simulink model "Visualization_MVP_AI"  (R2026b)
settings: Solver=ode4  StopTime=90  FixedStep=0.005
libraries: uavutilslib x1
settings Model: DataDictionary=QuadInterfaces_AI.sldd  Creator=JonathanTee  LastModifiedBy=JonathanTee

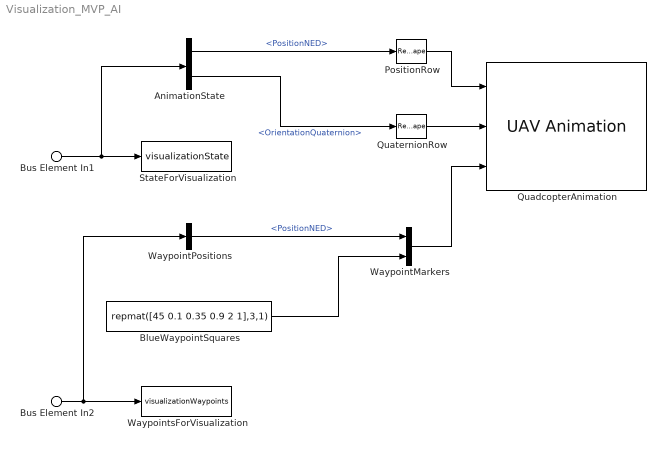
== system Visualization_MVP_AI ==
  Bus Element In1 : Inport  PortName=VehicleState
  Bus Element In2 : Inport  Port=2  PortName=WaypointTargets
  AnimationState : BusSelector  OutputSignals=PositionNED,OrientationQuaternion
  BlueWaypointSquares : Constant  Value=repmat([45 0.1 0.35 0.9 2 1],3,1)
  PositionRow : Reshape  OutputDimensionality=Row vector (2-D)
  QuadcopterAnimation : uavutilslib/UAV Animation  NumUAV=1  DynamicUAVConfig=off  UAVType=Multirotor  UAVSize=0.8  UAVColor=[0.9 0.05 0.04]  UAVTrajectoryAlpha=1  AlwaysShowAnimation=on  AxisLimits=[-0.8 2.8;-0.8 2.8;-0.25 2.8]  TrajectoryBufferSize=100000  InertialZDirection=Down  RotationFormat=Quaternion  DrawMarkers=on  SampleTime=0.05
  QuaternionRow : Reshape  OutputDimensionality=Row vector (2-D)
  StateForVisualization : ToWorkspace  VariableName=visualizationState  SaveFormat=Timeseries  SampleTime=-1
  WaypointMarkers : Concatenate  Mode=Multidimensional array  ConcatenateDimension=2
  WaypointPositions : BusSelector  OutputSignals=PositionNED
  WaypointsForVisualization : ToWorkspace  VariableName=visualizationWaypoints  SaveFormat=Timeseries  SampleTime=-1
  wires:
  WaypointMarkers/1 -> QuadcopterAnimation/3
  BlueWaypointSquares/1 -> WaypointMarkers/2
  WaypointPositions/1 -> WaypointMarkers/1  "<PositionNED>"
  QuaternionRow/1 -> QuadcopterAnimation/2
  PositionRow/1 -> QuadcopterAnimation/1
  AnimationState/2 -> QuaternionRow/1  "<OrientationQuaternion>"
  AnimationState/1 -> PositionRow/1  "<PositionNED>"
  Bus Element In1/1 -> StateForVisualization/1, AnimationState/1
  Bus Element In2/1 -> WaypointsForVisualization/1, WaypointPositions/1
